simulink model "HPP_Digital_Twin_Model"  (R2023b)
settings: Solver=VariableStepAuto  StartTime=0.0  StopTime=86400  RelTol=1e-3
settings Model: Creator=Duran  LastModifiedBy=Duran

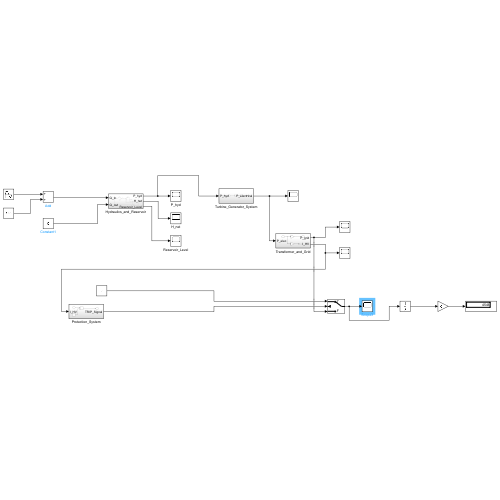
[thumbnail: Simulink's stored preview of the top-level diagram]
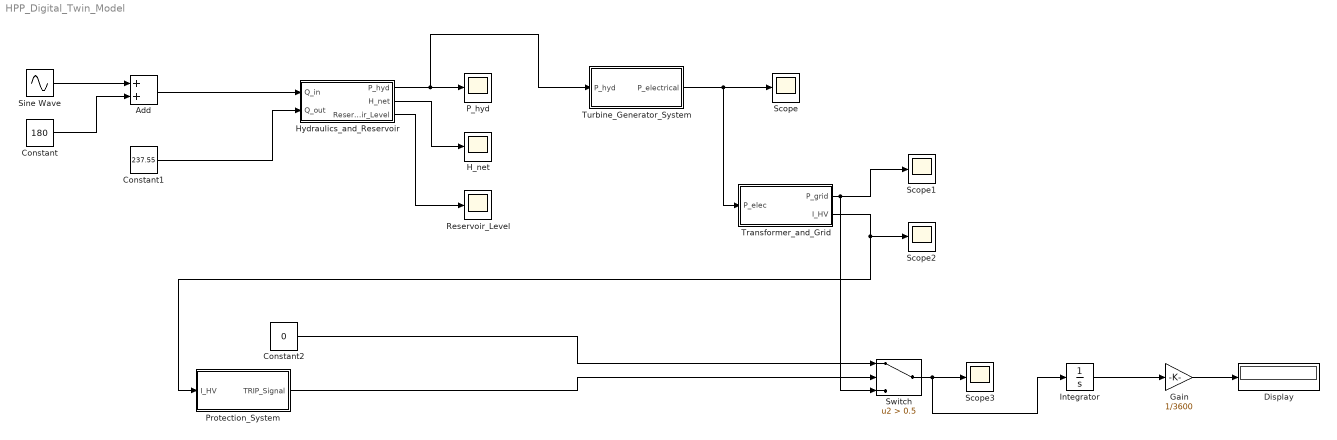
== system HPP_Digital_Twin_Model ==
  Add : Sum
  Constant : Constant  Value=180
  Constant1 : Constant  Value=237.55
  Constant2 : Constant  Value=0
  Display : Display
  Gain : Gain  Gain=1/3600
  H_net : Scope
  Hydraulics_and_Reservoir : Subsystem
  Integrator : Integrator
  P_hyd : Scope
  Protection_System : Subsystem
  Reservoir_Level : Scope
  Scope{,1..3} (4 alike) : Scope
  Sine Wave : Sin  Amplitude=20  Frequency=2*pi/86400  SampleTime=0
  Switch : Switch  Criteria=u2 > Threshold  Threshold=0.5  SaturateOnIntegerOverflow=off  InputSameDT=off
  Transformer_and_Grid : Subsystem
  Turbine_Generator_System : Subsystem
  wires:
  Sine Wave/1 -> Add/1
  Constant/1 -> Add/2
  Add/1 -> Hydraulics_and_Reservoir/1(Q_in)
  Constant1/1 -> Hydraulics_and_Reservoir/2(Q_out)
  Hydraulics_and_Reservoir/1(P_hyd) -> Turbine_Generator_System/1(P_hyd), P_hyd/1
  Hydraulics_and_Reservoir/2(H_net) -> H_net/1
  Hydraulics_and_Reservoir/3(Reservoir_Level) -> Reservoir_Level/1
  Turbine_Generator_System/1(P_electrical) -> Transformer_and_Grid/1(P_elec), Scope/1
  Transformer_and_Grid/1(P_grid) -> Switch/3, Scope1/1
  Transformer_and_Grid/2(I_HV) -> Protection_System/1(I_HV), Scope2/1
  Constant2/1 -> Switch/1
  Protection_System/1(TRIP_Signal) -> Switch/2
  Switch/1 -> Integrator/1, Scope3/1
  Integrator/1 -> Gain/1
  Gain/1 -> Display/1

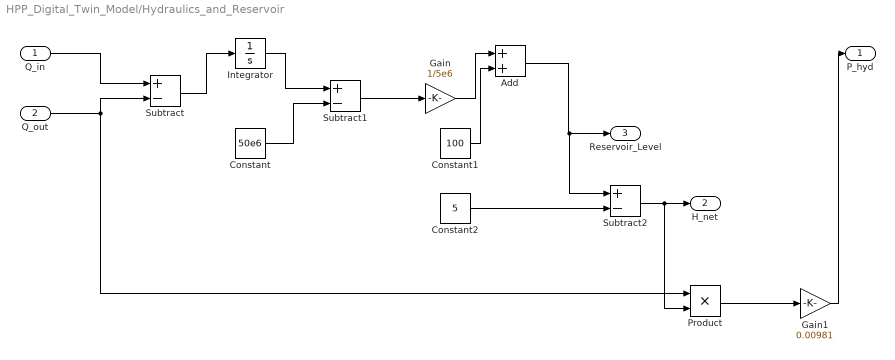
== system HPP_Digital_Twin_Model/Hydraulics_and_Reservoir ==
  Q_in : Inport
  Q_out : Inport  Port=2
  Add : Sum
  Constant : Constant  Value=50e6
  Constant1 : Constant  Value=100
  Constant2 : Constant  Value=5
  Gain : Gain  Gain=1/5e6
  Gain1 : Gain  Gain=0.00981
  Integrator : Integrator  InitialCondition=50e6
  Product : Product
  Subtract : Sum  Inputs=+-
  Subtract1 : Sum  Inputs=+-
  Subtract2 : Sum  Inputs=+-
  P_hyd : Outport
  H_net : Outport  Port=2
  Reservoir_Level : Outport  Port=3
  wires:
  Q_in/1 -> Subtract/1
  Q_out/1 -> Product/1, Subtract/2
  Subtract/1 -> Integrator/1
  Integrator/1 -> Subtract1/1
  Constant/1 -> Subtract1/2
  Subtract1/1 -> Gain/1
  Gain/1 -> Add/1
  Constant1/1 -> Add/2
  Add/1 -> Subtract2/1, Reservoir_Level/1
  Constant2/1 -> Subtract2/2
  Subtract2/1 -> Product/2, H_net/1
  Product/1 -> Gain1/1
  Gain1/1 -> P_hyd/1

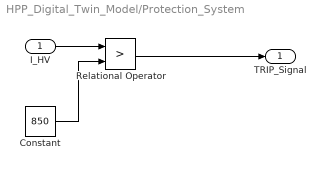
== system HPP_Digital_Twin_Model/Protection_System ==
  I_HV : Inport
  Constant : Constant  Value=850
  Relational Operator : RelationalOperator  Operator=>  OutDataTypeStr=boolean  RndMeth=Simplest  InputSameDT=off
  TRIP_Signal : Outport
  wires:
  I_HV/1 -> Relational Operator/1
  Constant/1 -> Relational Operator/2
  Relational Operator/1 -> TRIP_Signal/1

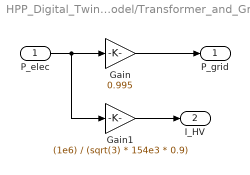
== system HPP_Digital_Twin_Model/Transformer_and_Grid ==
  P_elec : Inport
  Gain : Gain  Gain=0.995
  Gain1 : Gain  Gain=(1e6) / (sqrt(3) * 154e3 * 0.9)
  P_grid : Outport
  I_HV : Outport  Port=2
  wires:
  P_elec/1 -> Gain1/1, Gain/1
  Gain/1 -> P_grid/1
  Gain1/1 -> I_HV/1

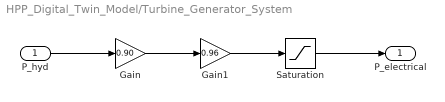
== system HPP_Digital_Twin_Model/Turbine_Generator_System ==
  P_hyd : Inport
  Gain : Gain  Gain=0.90
  Gain1 : Gain  Gain=0.96
  Saturation : Saturate  UpperLimit=191.28  LowerLimit=0
  P_electrical : Outport
  wires:
  P_hyd/1 -> Gain/1
  Gain/1 -> Gain1/1
  Gain1/1 -> Saturation/1
  Saturation/1 -> P_electrical/1
